simulink model "clockstudy"  (Simulink 4.00)
settings: Solver=FixedStepDiscrete  StartTime=0.0  StopTime=12.0  FixedStep=1  RelTol=1e-3
settings Model: Creator=mcar  LastModifiedBy=mcar  OptimizeBlockIOStorage=off  BlockReductionOpt=off

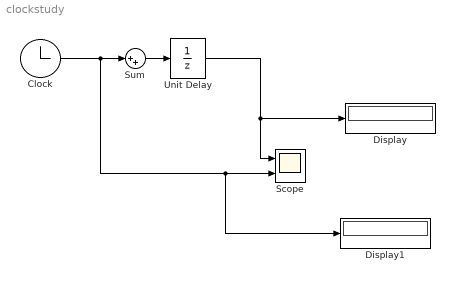
== system clockstudy ==
  Clock : Clock
      settings: Decimation=100
  Display : Display
      settings: Format=short
  Display1 : Display
      settings: Format=short
  Scope : Scope  NumInputPorts=2
      settings: TimeRange=auto  YMin=-5~-5  YMax=5~5  SaveToWorkspace=off  SaveName=ScopeData  LimitDataPoints=on  MaxDataPoints=5000
  Sum : Sum  Inputs=|++  SaturateOnIntegerOverflow=on
  Unit Delay : UnitDelay  X0=0  SampleTime=1
  wires:
  Clock/1 -> Scope/2, Display1/1, Sum/1
  Unit Delay/1 -> Scope/1, Display/1
  Sum/1 -> Unit Delay/1
